simulink subsystem "ctrl_CS2"  (R2025b)
settings: Solver=VariableStepAuto  StartTime=0.0  StopTime=10.0  RelTol=1e-3
values from neighbouring files (symbols this model uses):
  A = [1 0 0 0 2.70127656662e-05 1.00008362958 0.0539210392304 0.167052905048 0.000996918625491 -3.04176177404e-06 0.993845368835 -0.00607175725634 ... (16 elements, 4x4)]    [data_test_01.mat]    (also in qube_model.m = sys_dt.A)
  alpha_sign = -1    [Hardware_settings.m]    (also in data_test_01.mat; params_CS2.m = 1)
  B = [9.00986698557e-06 8.89404027496e-06 0.0179959975588 0.0177536761881]    [data_test_01.mat]    (also in qube_model.m = sys_dt.B)
  C = [1  0  0  0; 0  1  0  0]    [data_test_01.mat]    (also in qube_model.m = sys_dt.C)
  F = [-19.3998122063 110.195195868 -5.59381147179 8.15976877824]    [data_test_01.mat]    (also in params_CS2.m = place(A, B, exp(ps*ts)))
  Fi = -14.922072369    [data_test_01.mat]    (also in params_CS2.m = 0)
  int_band = 0.0349065850399    [data_test_01.mat]    (also in params_CS2.m = 0.0872664625997)
  Lo = [0.179270844532  -0.00612381249307; -0.0107164751417  0.18077545229; 7.51704343687  -0.62814538936; -1.44329109342  7.88868722606]    [data_test_01.mat]    (also in params_CS2.m = place(A', C', po_z)')
  ref_tau = 0.2    [data_test_01.mat]    (also in params_CS2.m)
  ts = 1/1000    (= 0.001)    [Hardware_settings.m]    (also in data_test_01.mat; qube_model.m)
  u_max = 10    [data_test_01.mat]    (also in params_CS2.m)
  xhat0_offset = [0 0 0 0]    [data_test_01.mat]    (also in params_CS2.m = [0; 0; 0; 0])
settings Model: Creator=jaylen  LastModifiedBy=jaylen

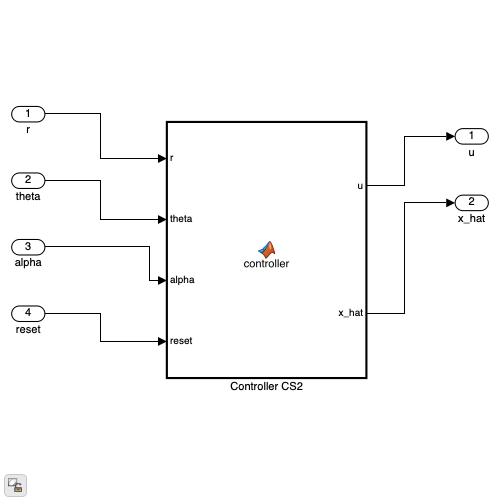
[thumbnail: Simulink's stored preview of the top-level diagram]
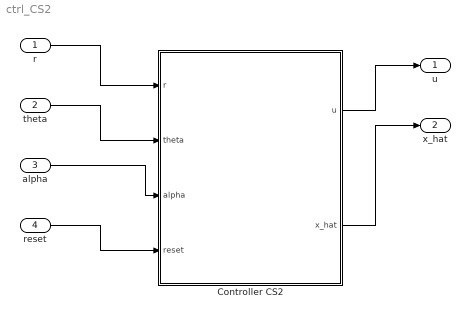
== system ctrl_CS2 ==
  r : Inport
  theta : Inport  Port=2
  alpha : Inport  Port=3
  reset : Inport  Port=4
  Controller CS2 : MATLAB Function  TreatAsAtomicUnit=on
  u : Outport
  x_hat : Outport  Port=2
  wires:
  Controller CS2/1(u) -> u/1
  Controller CS2/2(x_hat) -> x_hat/1
  r/1 -> Controller CS2/1(r)
  theta/1 -> Controller CS2/2(theta)
  alpha/1 -> Controller CS2/3(alpha)
  reset/1 -> Controller CS2/4(reset)

== matlab function ctrl_CS2/Controller CS2 ==
  settings: updateMethod=DISCRETE  sampleTime=ts
  data: r input; u output; theta input; alpha input; reset input; x_hat output; F parameter; Fi parameter; Lo parameter; A parameter; B parameter; C parameter; ts parameter; ref_tau parameter; int_band parameter; xhat0_offset parameter; u_max parameter; alpha_sign parameter
function [u, x_hat] = controller(r, theta, alpha, reset, F, Fi, Lo, A, B, C, ts, ref_tau, int_band, xhat0_offset, u_max, alpha_sign)
%CONTROLLER Discrete-time SFC with integral action and a Luenberger observer (CS2).
% Every stage of the control system is in this one block (Task 5 rule):
%   1. Reference filter:  r_f(k+1) = r_f(k) + ts/ref_tau (r - r_f(k)),  x* = [r_f; 0; 0; 0], u* = 0
%   2. Integral action:   x_i(k+1) = x_i(k) + ts (theta(k) - r), only while |theta - r| <= int_band
%                         and the voltage isn't limited (anti-windup)
%   3. Control law:       u(k) = -F (x_hat(k) - x*) - Fi x_i(k) + u*, limited to +/-u_max
%   4. Observer:          x_hat(k+1) = A x_hat(k) + B u(k) + Lo (y(k) - C x_hat(k))
% The observer is updated with the limited voltage that actually reaches the
% motor. When the controller is enabled, the observer starts from the measured
% angles with zero velocities, the reference filter from the measured theta and
% the integral from zero; xhat0_offset adds an initial estimation error for
% showing observer convergence in simulation (keep it zero on the hardware).
% Set Fi = 0 to run without integral action, or ref_tau = 0 to skip the filter.
% Inputs: r, theta, alpha in rad; reset = 1 (controller disabled) restarts all
% states and holds u at 0. Outputs: u, the motor voltage Vm in V; x_hat.
% alpha_sign corrects the pendulum encoder's direction: +1 in simulation (the
% plant models use the model convention), -1 on the QUBE (set in Hardware_settings.m).
%#codegen

alpha = alpha_sign*alpha;

persistent xh xi rf
y = [theta; alpha];
if isempty(xh) || reset
    xh = [y; 0; 0] + xhat0_offset;
    xi = 0;
    rf = theta;
end
x_hat = xh;

% 1. Reference filter
if ref_tau > 0
    rf = rf + ts/ref_tau*(r - rf);
else
    rf = r;
end
x_ref = [rf; 0; 0; 0];
u_ref = 0;

% 3. Control law, with the amplifier limit
u_unlimited = -F*(xh - x_ref) - Fi*xi + u_ref;
u = min(max(u_unlimited, -u_max), u_max);
if reset
    u = 0;
end

% 2. Integral of the arm error, conditional and with anti-windup
e = theta - r;
dxi = ts*e;
winding_up = (u_unlimited > u_max && -Fi*dxi > 0) || (u_unlimited < -u_max && -Fi*dxi < 0);
if abs(e) <= int_band && ~winding_up && ~reset
    xi = xi + dxi;
end

% 4. Observer
xh = A*xh + B*u + Lo*(y - C*xh);
end
